simulink model "part1_dc_motor"  (R2024b)
settings: Solver=ode45  StartTime=0.0  StopTime=2  MaxStep=0.002  RelTol=1e-8  AbsTol=1e-10
model workspace (MAT data in the model file):
  J = 0.01
  KT = 0.2
  Ke = 0.2
  La = 0.05
  Ra = 2
  d1 = 0.01
  d2 = 0.005
  ia0 = 0
  omega0 = 0
  theta0 = 0
settings Model: Creator=matiasgarcia  LastModifiedBy=matiasgarcia
settings DataIOCC: SaveOutput=off  SignalLogging=off  SaveTime=off

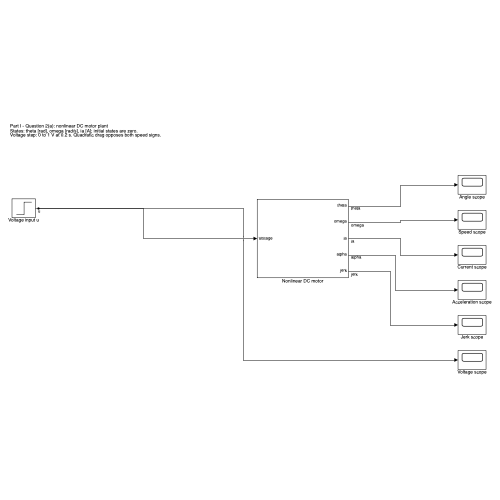
[thumbnail: Simulink's stored preview of the top-level diagram]
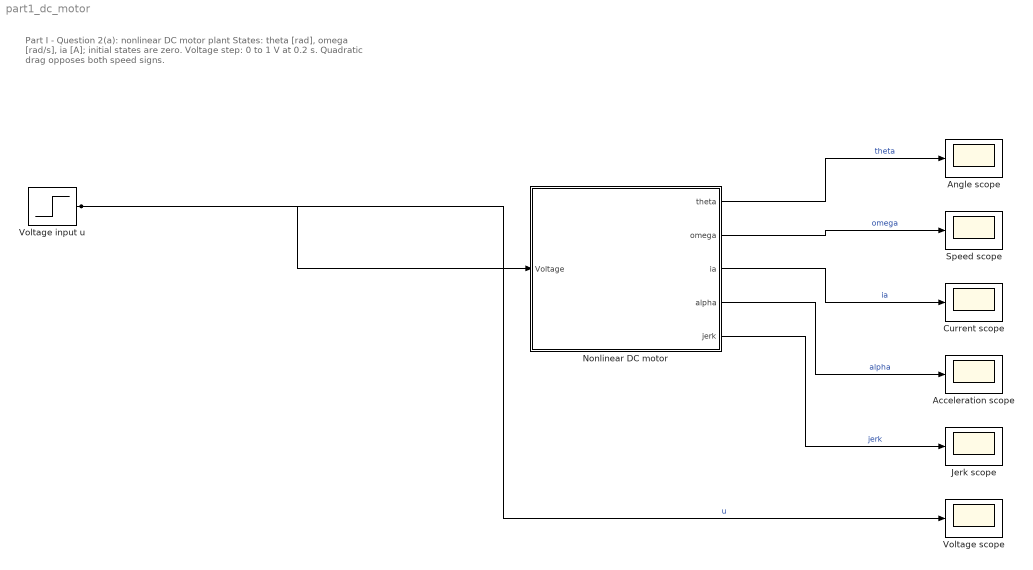
== system part1_dc_motor ==
  note: Part I - Question 2(a): nonlinear DC motor plant
      | States: theta [rad], omega [rad/s], ia [A]; initial states are zero.
      | Voltage step: 0 to 1 V at 0.2 s. Quadratic drag opposes both speed signs.
  Acceleration scope : Scope
  Angle scope : Scope
  Current scope : Scope
  Jerk scope : Scope
  Nonlinear DC motor : Subsystem
  Speed scope : Scope
  Voltage input u : Step  Time=0.2  SampleTime=0
  Voltage scope : Scope
  wires:
  Voltage input u/1 -> Nonlinear DC motor/1(Voltage), Voltage scope/1  "u"
  Nonlinear DC motor/1(theta) -> Angle scope/1  "theta"
  Nonlinear DC motor/2(omega) -> Speed scope/1  "omega"
  Nonlinear DC motor/3(ia) -> Current scope/1  "ia"
  Nonlinear DC motor/4(alpha) -> Acceleration scope/1  "alpha"
  Nonlinear DC motor/5(jerk) -> Jerk scope/1  "jerk"

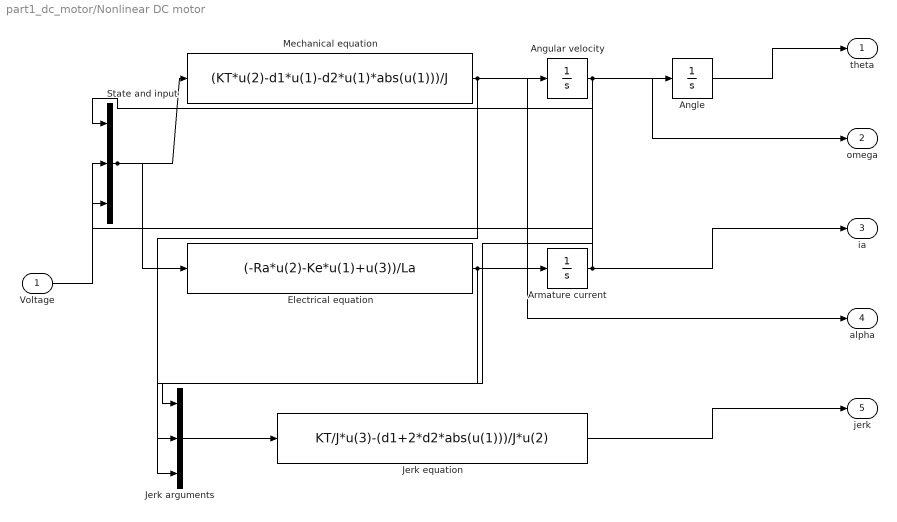
== system part1_dc_motor/Nonlinear DC motor ==
  Voltage : Inport
  Angle : Integrator  InitialCondition=theta0
  Angular velocity : Integrator  InitialCondition=omega0
  Armature current : Integrator  InitialCondition=ia0
  Electrical equation : Fcn  Expr=(-Ra*u(2)-Ke*u(1)+u(3))/La
  Jerk arguments : Mux  Inputs=3
  Jerk equation : Fcn  Expr=KT/J*u(3)-(d1+2*d2*abs(u(1)))/J*u(2)
  Mechanical equation : Fcn  Expr=(KT*u(2)-d1*u(1)-d2*u(1)*abs(u(1)))/J
  State and input : Mux  Inputs=3
  theta : Outport
  omega : Outport  Port=2
  ia : Outport  Port=3
  alpha : Outport  Port=4
  jerk : Outport  Port=5
  wires:
  Angular velocity/1 -> State and input/1, Angle/1, Jerk arguments/1, omega/1
  Armature current/1 -> State and input/2, ia/1
  Voltage/1 -> State and input/3
  State and input/1 -> Mechanical equation/1, Electrical equation/1
  Mechanical equation/1 -> Angular velocity/1, Jerk arguments/2, alpha/1
  Electrical equation/1 -> Armature current/1, Jerk arguments/3
  Jerk arguments/1 -> Jerk equation/1
  Angle/1 -> theta/1
  Jerk equation/1 -> jerk/1
